simulink model "ftGrid_N5_RL"  (R2026a)
settings: Solver=ode1  StopTime=12  FixedStep=1e-3
libraries: ee_lib x29, nesl_utility x20, fl_lib x6
settings Model: Creator=kjaer  LastModifiedBy=kjaer

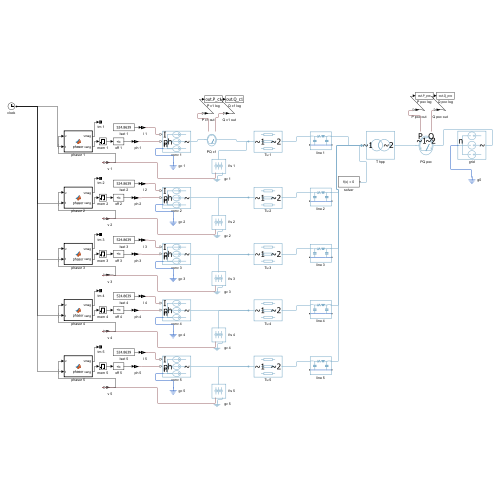
[thumbnail: Simulink's stored preview of the top-level diagram]
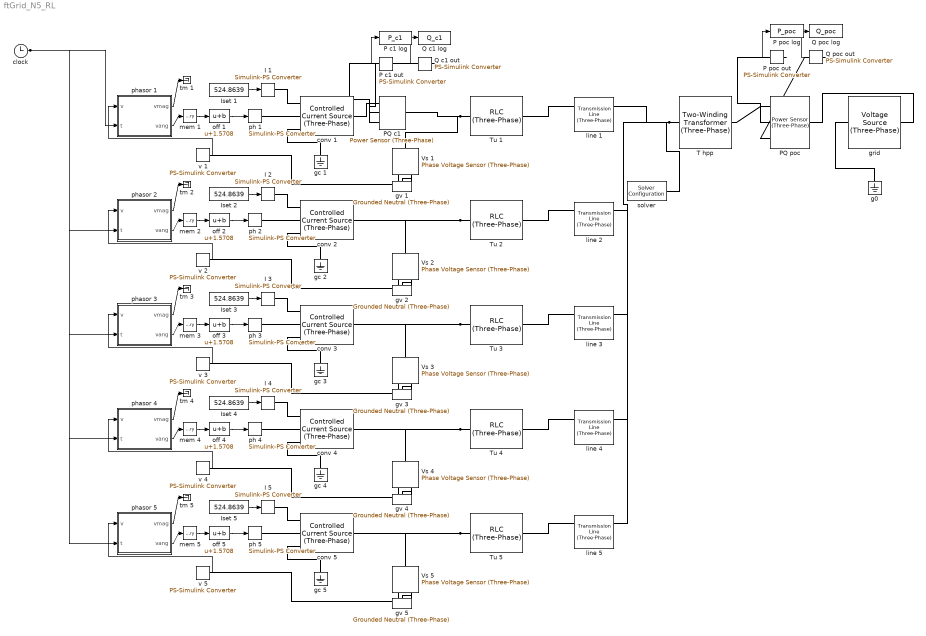
== system ftGrid_N5_RL ==
  I {1..5} (5 alike) : nesl_utility/Simulink-PS Converter  PhysicalDomain=network_engine_domain  SubClassName=ps_input  LeftPortType=input  RightPortType=output  PseudoPeriodic=off  Frequencies=[]  NoiseDistribution=none  NoiseParameters=[]  Unit=A  AffineConversion=off  FilteringAndDerivatives=provide  SimscapeFilterOrder=1  InputFilterTimeConstant=0.001  UdotUserProvided=0
  Iset {1..5} (5 alike) : Constant  Value=524.8639
  P c1 log : ToWorkspace  VariableName=P_c1  SaveFormat=Timeseries  SampleTime=-1
  P c1 out : nesl_utility/PS-Simulink Converter  PhysicalDomain=network_engine_domain  SubClassName=ps_output  LeftPortType=input  RightPortType=output  PseudoPeriodic=off  Frequencies=[]  VectorFormat=inherit  Unit=inherit  AffineConversion=off
  P poc log : ToWorkspace  VariableName=P_poc  SaveFormat=Timeseries  SampleTime=-1
  P poc out : nesl_utility/PS-Simulink Converter  PhysicalDomain=network_engine_domain  SubClassName=ps_output  LeftPortType=input  RightPortType=output  PseudoPeriodic=off  Frequencies=[]  VectorFormat=inherit  Unit=inherit  AffineConversion=off
  PQ c1 : ee_lib/Sensors & Transducers/Power Sensor (Three-Phase)  port_option=ee.enum.threePhasePort.composite  load_type=ee.enum.passive.type_balanced.balanced  f0=50 Hz
  PQ poc : ee_lib/Sensors & Transducers/Power Sensor (Three-Phase)  port_option=ee.enum.threePhasePort.composite  load_type=ee.enum.passive.type_balanced.balanced  f0=50 Hz
  Q c1 log : ToWorkspace  VariableName=Q_c1  SaveFormat=Timeseries  SampleTime=-1
  Q c1 out : nesl_utility/PS-Simulink Converter  PhysicalDomain=network_engine_domain  SubClassName=ps_output  LeftPortType=input  RightPortType=output  PseudoPeriodic=off  Frequencies=[]  VectorFormat=inherit  Unit=inherit  AffineConversion=off
  Q poc log : ToWorkspace  VariableName=Q_poc  SaveFormat=Timeseries  SampleTime=-1
  Q poc out : nesl_utility/PS-Simulink Converter  PhysicalDomain=network_engine_domain  SubClassName=ps_output  LeftPortType=input  RightPortType=output  PseudoPeriodic=off  Frequencies=[]  VectorFormat=inherit  Unit=inherit  AffineConversion=off
  T hpp : ee_lib/Passive/Transformers/Two-Winding Transformer (Three-Phase)  SRated=250e6 A*V  FRated=50 Hz  Winding1Connection=ee.enum.windingconnection.Yg  VRated1=33e3 V  Winding2Connection=ee.enum.windingconnection.Yg  VRated2=132e3 V  CoreType=ee.enum.coretype.threelimb  pu_Rw1=0.0015  pu_Rw2=0.0015  leakage_reactance_option=ee.enum.transformer_leakage.include  pu_Xl1=0.06  pu_Xl2=0.06  magnetizing_resistance_option=ee.enum.transformer_magnetizingResistance.include  pu_Rm=500  magnetizing_reactance_option=ee.enum.transformer_magnetizingReactance.include  saturation_option=ee.enum.transformer_saturation.exclude  pu_Xm=500  current_data=[0, .002, 1, 2]  magnetic_flux_data=[0, 1.2, 1.5, 1.51]  pu_X0=0.5  i1_specify=off  i1_priority=None  i1=[0, 0, 0] A  i1_nominal_specify=off  i1_nominal_value=1  i1_nominal_unit=A  i2_specify=off  i2_priority=None  i2=[0, 0, 0] A  i2_nominal_specify=off  i2_nominal_value=1  i2_nominal_unit=A  phi_specify=off  phi_priority=None  phi=[0, 0, 0]  phi_nominal_specify=off  phi_nominal_value=1  phi_nominal_unit=1
  Tu {1..5} (5 alike) : ee_lib/Passive/RLC Assemblies/RLC (Three-Phase)  port_option=ee.enum.threePhasePort.composite  component_structure=ee.enum.rlc.structure.SeriesRL  R=0.264 Ohm  L=0.0063025 H  C=1e-6 F  R_parasitic=0 Ohm  G_parasitic=0 1/Ohm  IL_specify=off  IL_priority=High  IL=[0, 0, 0] A  IL_nominal_specify=off  IL_nominal_value=1  IL_nominal_unit=A  VC_specify=off  VC_priority=High  VC=[0, 0, 0] V  VC_nominal_specify=off  VC_nominal_value=1  VC_nominal_unit=V
  Vs {1..5} (5 alike) : ee_lib/Sensors & Transducers/Phase Voltage Sensor (Three-Phase)  port_option=ee.enum.threePhasePort.composite
  clock : Clock
  conv {1..5} (5 alike) : ee_lib/Sources/Controlled Current Source (Three-Phase)  port_option=ee.enum.threePhasePort.composite  input_option=ee.enum.inputType.singleFreqAC  FRated=50 Hz  G_parasitic=0 1/Ohm
  g0 : fl_lib/Electrical/Electrical Elements/Electrical Reference
  gc {1..5} (5 alike) : fl_lib/Electrical/Electrical Elements/Electrical Reference
  grid : ee_lib/Sources/Voltage Source (Three-Phase)  vline_rms=132e3 V  shift=0 deg  freq=50 Hz  impedance_option=1  SShortCircuit=1800e6 A*V  XR=10  R=0.01 Ohm  L=3.97e-4 H  harmonic_option=0  harmonic_orders=[5, 7, 11, 13]  harmonic_ratios=[.1, .1, .1, .1]  G_parasitic=0 1/Ohm  I_specify=off  I_priority=None  I=[0, 0, 0] A  I_nominal_specify=off  I_nominal_value=1  I_nominal_unit=A
  gv {1..5} (5 alike) : ee_lib/Connectors & References/Grounded Neutral (Three-Phase)  port_option=ee.enum.threePhasePort.composite
  line {1..5} (5 alike) : ee_lib/Passive/Lines/Transmission Line (Three-Phase)  port_option=ee.enum.threePhasePort.composite  length=2 km  freq=50 Hz  prm=ee.enum.lines.parameterization3ph.posZeroSeqParam  R=0.02 Ohm/km  Rm=0 Ohm/km  L=0.5 mH/km  M=0.1 mH/km  Cl=0.3 uF/km  Cg=0.1 uF/km  Rpos=0.10 Ohm/km  Rzero=0.3 Ohm/km  Lpos=0.38 mH/km  Lzero=1.2 mH/km  Cpos=0.25 uF/km  Czero=0.20 uF/km  ModelTwoSections=ee.enum.enable.no  N=1  InterfacePosition=0.5 km  N1sec=1  N2sec=1  Access_ground=ee.enum.enable.no  R_parasitic=1e-6 Ohm  G_parasitic=1e-6 1/Ohm
  mem {1..5} (5 alike) : Memory
  off {1..5} (5 alike) : Bias  Bias=1.5708  SaturateOnIntegerOverflow=off
  ph {1..5} (5 alike) : nesl_utility/Simulink-PS Converter  PhysicalDomain=network_engine_domain  SubClassName=ps_input  LeftPortType=input  RightPortType=output  PseudoPeriodic=off  Frequencies=[]  NoiseDistribution=none  NoiseParameters=[]  Unit=rad  AffineConversion=off  FilteringAndDerivatives=provide  SimscapeFilterOrder=1  InputFilterTimeConstant=0.001  UdotUserProvided=0
  phasor 1 : MATLAB Function  TreatAsAtomicUnit=on
  phasor 2 : MATLAB Function  TreatAsAtomicUnit=on
  phasor 3 : MATLAB Function  TreatAsAtomicUnit=on
  phasor 4 : MATLAB Function  TreatAsAtomicUnit=on
  phasor 5 : MATLAB Function  TreatAsAtomicUnit=on
  solver : nesl_utility/Solver Configuration  PhysicalDomain=network_engine_domain  SubClassName=solver  LeftPortType=input  RightPortType=generic  Tones=[]  Harmonics=[]  SimulateNoise=off  Profile=off  UseLocalSampling=off  EnableSwitchedLinearOptims=on  FrequencyDomain=off  UseCCode=off  RelTol=0.001  AbsTol=0.001  MinStep=1e-09  ToWorkspace=off  RevertToSquareIcSolve=off  NumHomotopyIterations=100  PhasorMode=off  PhasorModeNumHarmonics=1  ConsistencySolver=NEWTON_XTOL_AFTER_FTOL  CanonicalOrdering=CANONICAL  OptimizeIntermediates=OPTIMIZED  IndexReductionMethod=DerivativeReplacement  DoDC=off  ResidualTolerance=1e-09  ConsistencyTolSource=GLOBAL  ConsistencyAbsTol=0.001  ConsistencyRelTol=0.001  ConsistencyTolFactor=0.001  UseLocalSolver=on  LocalSolverChoice=NE_BACKWARD_EULER_ADVANCER  ResolveIndetEquations=on  FunctionEvalNumThread=1  LocalSolverSampleTime=1e-3  DoFixedCost=on  MaxNonlinIter=1  MaxModeIter=2  ComputeImpulses=off  ImpulseIterations=2  LinearAlgebra=auto  LinearAlgebraNumThread=0  EquationFormulation=NE_FREQUENCY_TIME_EF  DelaysMemoryBudget=1024  AutomaticFiltering=on  FilteringTimeConstant=0.001  PartitionStorageMethod=AS_NEEDED  PartitionMemoryBudget=1024  PartitionMethod=ROBUST  MultibodyUseLocalSolver=off  MultibodyLocalSolverChoice=ODE1  MultibodyLocalSolverSampleTime=0.001
  tm {1..5} (5 alike) : Terminator
  v {1..5} (5 alike) : nesl_utility/PS-Simulink Converter  PhysicalDomain=network_engine_domain  SubClassName=ps_output  LeftPortType=input  RightPortType=output  PseudoPeriodic=off  Frequencies=[]  VectorFormat=inherit  Unit=inherit  AffineConversion=off
  wires:
  P poc out/1 -> P poc log/1
  Q poc out/1 -> Q poc log/1
  P c1 out/1 -> P c1 log/1
  Q c1 out/1 -> Q c1 log/1
  v 1/1 -> phasor 1/1(v)
  clock/1 -> phasor 1/2(t), phasor 2/2(t), phasor 3/2(t), phasor 4/2(t), phasor 5/2(t)
  phasor 1/2(vang) -> mem 1/1
  mem 1/1 -> off 1/1
  off 1/1 -> ph 1/1
  Iset 1/1 -> I 1/1
  phasor 1/1(vmag) -> tm 1/1
  v 2/1 -> phasor 2/1(v)
  phasor 2/2(vang) -> mem 2/1
  mem 2/1 -> off 2/1
  off 2/1 -> ph 2/1
  Iset 2/1 -> I 2/1
  phasor 2/1(vmag) -> tm 2/1
  v 3/1 -> phasor 3/1(v)
  phasor 3/2(vang) -> mem 3/1
  mem 3/1 -> off 3/1
  off 3/1 -> ph 3/1
  Iset 3/1 -> I 3/1
  phasor 3/1(vmag) -> tm 3/1
  v 4/1 -> phasor 4/1(v)
  phasor 4/2(vang) -> mem 4/1
  mem 4/1 -> off 4/1
  off 4/1 -> ph 4/1
  Iset 4/1 -> I 4/1
  phasor 4/1(vmag) -> tm 4/1
  v 5/1 -> phasor 5/1(v)
  phasor 5/2(vang) -> mem 5/1
  mem 5/1 -> off 5/1
  off 5/1 -> ph 5/1
  Iset 5/1 -> I 5/1
  phasor 5/1(vmag) -> tm 5/1
  connections:
  grid/LConn1 -- g0/LConn1
  grid/RConn1 -- PQ poc/RConn1
  PQ poc/LConn1 -- T hpp/RConn1
  solver/RConn1 -- line 1/RConn1 -- line 2/RConn1 -- line 3/RConn1 -- line 4/RConn1 -- T hpp/LConn1 -- line 5/RConn1
  PQ poc/LConn2 -- P poc out/LConn1
  PQ poc/LConn3 -- Q poc out/LConn1
  line 1/LConn1 -- Tu 1/RConn1
  conv 1/RConn1 -- PQ c1/LConn1
  Tu 1/LConn1 -- PQ c1/RConn1 -- Vs 1/LConn1
  PQ c1/LConn2 -- P c1 out/LConn1
  PQ c1/LConn3 -- Q c1 out/LConn1
  conv 1/LConn3 -- gc 1/LConn1
  Vs 1/RConn2 -- gv 1/LConn1
  Vs 1/RConn1 -- v 1/LConn1
  I 1/RConn1 -- conv 1/LConn1
  ph 1/RConn1 -- conv 1/LConn2
  line 2/LConn1 -- Tu 2/RConn1
  Tu 2/LConn1 -- conv 2/RConn1 -- Vs 2/LConn1
  conv 2/LConn3 -- gc 2/LConn1
  Vs 2/RConn2 -- gv 2/LConn1
  Vs 2/RConn1 -- v 2/LConn1
  I 2/RConn1 -- conv 2/LConn1
  ph 2/RConn1 -- conv 2/LConn2
  line 3/LConn1 -- Tu 3/RConn1
  Tu 3/LConn1 -- conv 3/RConn1 -- Vs 3/LConn1
  conv 3/LConn3 -- gc 3/LConn1
  Vs 3/RConn2 -- gv 3/LConn1
  Vs 3/RConn1 -- v 3/LConn1
  I 3/RConn1 -- conv 3/LConn1
  ph 3/RConn1 -- conv 3/LConn2
  line 4/LConn1 -- Tu 4/RConn1
  Tu 4/LConn1 -- conv 4/RConn1 -- Vs 4/LConn1
  conv 4/LConn3 -- gc 4/LConn1
  Vs 4/RConn2 -- gv 4/LConn1
  Vs 4/RConn1 -- v 4/LConn1
  I 4/RConn1 -- conv 4/LConn1
  ph 4/RConn1 -- conv 4/LConn2
  line 5/LConn1 -- Tu 5/RConn1
  Tu 5/LConn1 -- conv 5/RConn1 -- Vs 5/LConn1
  conv 5/LConn3 -- gc 5/LConn1
  Vs 5/RConn2 -- gv 5/LConn1
  Vs 5/RConn1 -- v 5/LConn1
  I 5/RConn1 -- conv 5/LConn1
  ph 5/RConn1 -- conv 5/LConn2

== matlab function ftGrid_N5_RL/phasor 1 ==
  data: v input; vmag output; t input; vang output
function [vmag, vang] = phasor(v, t)
% space phasor of the phase voltages at a fixed 50 Hz: rms line voltage and angle
a = complex(-0.5, sqrt(3)/2);
s = 2/3*(v(1) + a*v(2) + a^2*v(3)) * exp(complex(0, -2*pi*50*t));
vmag = abs(s)*sqrt(3/2);
vang = angle(s);
end

== matlab function ftGrid_N5_RL/phasor 3 ==
  data: v input; vmag output; t input; vang output
function [vmag, vang] = phasor(v, t)
% space phasor of the phase voltages at a fixed 50 Hz: rms line voltage and angle
a = complex(-0.5, sqrt(3)/2);
s = 2/3*(v(1) + a*v(2) + a^2*v(3)) * exp(complex(0, -2*pi*50*t));
vmag = abs(s)*sqrt(3/2);
vang = angle(s);
end

== matlab function ftGrid_N5_RL/phasor 4 ==
  data: v input; vmag output; t input; vang output
function [vmag, vang] = phasor(v, t)
% space phasor of the phase voltages at a fixed 50 Hz: rms line voltage and angle
a = complex(-0.5, sqrt(3)/2);
s = 2/3*(v(1) + a*v(2) + a^2*v(3)) * exp(complex(0, -2*pi*50*t));
vmag = abs(s)*sqrt(3/2);
vang = angle(s);
end

== matlab function ftGrid_N5_RL/phasor 5 ==
  data: v input; vmag output; t input; vang output
function [vmag, vang] = phasor(v, t)
% space phasor of the phase voltages at a fixed 50 Hz: rms line voltage and angle
a = complex(-0.5, sqrt(3)/2);
s = 2/3*(v(1) + a*v(2) + a^2*v(3)) * exp(complex(0, -2*pi*50*t));
vmag = abs(s)*sqrt(3/2);
vang = angle(s);
end

== matlab function ftGrid_N5_RL/phasor 2 ==
  data: v input; vmag output; t input; vang output
function [vmag, vang] = phasor(v, t)
% space phasor of the phase voltages at a fixed 50 Hz: rms line voltage and angle
a = complex(-0.5, sqrt(3)/2);
s = 2/3*(v(1) + a*v(2) + a^2*v(3)) * exp(complex(0, -2*pi*50*t));
vmag = abs(s)*sqrt(3/2);
vang = angle(s);
end
